simulink model "pv_resource_dynamic_standalone"  (R2024b)
settings: Solver=ode14x  StartTime=0.0  StopTime=1.0  FixedStep=5e-5  RelTol=1e-3
InitFcn:
  | setup_v2_paths; define_resource_buses(true); V2=define_v2_parameters(false); V2.PV.dynamic.enabled=true; V2.PV.filter.topology='LCL';
undefined symbols (not defined in the file): DiscIntNeverNeededParam
libraries: nesl_utility x18, ee_lib x12, fl_lib x11
settings Model: SimulationMode=accelerator  Creator=qyj  LastModifiedBy=qyj

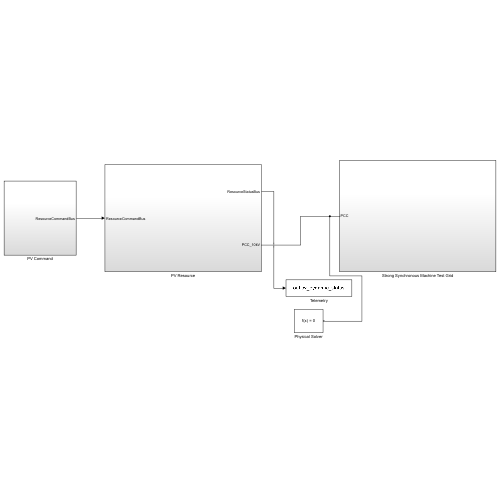
[thumbnail: Simulink's stored preview of the top-level diagram]
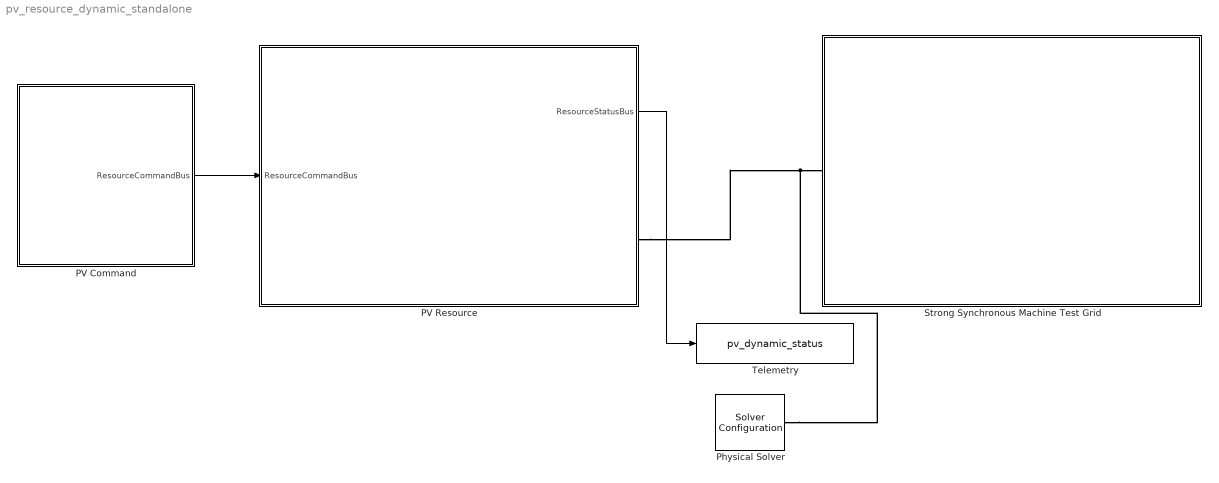
== system pv_resource_dynamic_standalone ==
  PV Command : Subsystem
  PV Resource : Subsystem
  Physical Solver : nesl_utility/Solver Configuration  PhysicalDomain=network_engine_domain  SubClassName=solver  LeftPortType=input  RightPortType=generic  Tones=[]  Harmonics=[]  SimulateNoise=off  Profile=off  UseLocalSampling=off  EnableSwitchedLinearOptims=on  FrequencyDomain=off  UseCCode=off  RelTol=0.001  AbsTol=0.001  MinStep=1e-09  ToWorkspace=off  RevertToSquareIcSolve=off  NumHomotopyIterations=100  PhasorMode=off  PhasorModeNumHarmonics=1  ConsistencySolver=NEWTON_XTOL_AFTER_FTOL  IndexReductionMethod=DerivativeReplacement  DoDC=off  ResidualTolerance=1e-09  ConsistencyTolSource=GLOBAL  ConsistencyAbsTol=0.001  ConsistencyRelTol=0.001  ConsistencyTolFactor=0.001  UseLocalSolver=off  LocalSolverChoice=NE_BACKWARD_EULER_ADVANCER  ResolveIndetEquations=on  FunctionEvalNumThread=1  LocalSolverSampleTime=0.001  DoFixedCost=off  MaxNonlinIter=3  MaxModeIter=2  ComputeImpulses=off  ImpulseIterations=2  LinearAlgebra=auto  LinearAlgebraNumThread=0  EquationFormulation=NE_TIME_EF  DelaysMemoryBudget=1024  AutomaticFiltering=on  FilteringTimeConstant=0.001  PartitionStorageMethod=AS_NEEDED  PartitionMemoryBudget=1024  PartitionMethod=ROBUST  MultibodyUseLocalSolver=off  MultibodyLocalSolverChoice=ODE1  MultibodyLocalSolverSampleTime=0.001
  Strong Synchronous Machine Test Grid : Subsystem
  Telemetry : ToWorkspace  VariableName=pv_dynamic_status  SaveFormat=Timeseries  SampleTime=-1
  wires:
  PV Command/1(ResourceCommandBus) -> PV Resource/1(ResourceCommandBus)
  PV Resource/1(ResourceStatusBus) -> Telemetry/1
  connections:
  PV Resource/RConn1 -- Strong Synchronous Machine Test Grid/LConn1 -- Physical Solver/RConn1

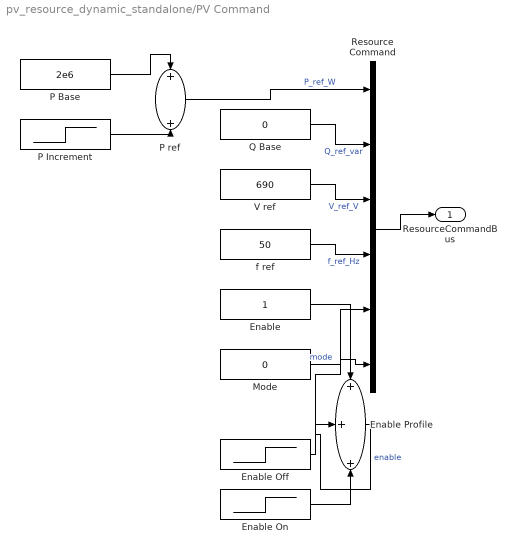
== system pv_resource_dynamic_standalone/PV Command ==
  Enable : Constant
  Enable Off : Step  Time=10  After=-1  SampleTime=0
  Enable On : Step  Time=11  SampleTime=0
  Enable Profile : Sum  Inputs=+++
  Mode : Constant  Value=0
  P Base : Constant  Value=2e6
  P Increment : Step  Time=0.3  After=1e6  SampleTime=0
  P ref : Sum
  Q Base : Constant  Value=0
  Resource Command : BusCreator  Inputs=6  OutDataTypeStr=Bus: ResourceCommandBus
  V ref : Constant  Value=690
  f ref : Constant  Value=50
  ResourceCommandBus : Outport
  wires:
  P Base/1 -> P ref/1
  P Increment/1 -> P ref/2
  Enable/1 -> Enable Profile/1
  Enable Off/1 -> Enable Profile/2
  Enable On/1 -> Enable Profile/3
  P ref/1 -> Resource Command/1  "P_ref_W"
  Q Base/1 -> Resource Command/2  "Q_ref_var"
  V ref/1 -> Resource Command/3  "V_ref_V"
  f ref/1 -> Resource Command/4  "f_ref_Hz"
  Enable Profile/1 -> Resource Command/5  "enable"
  Mode/1 -> Resource Command/6  "mode"
  Resource Command/1 -> ResourceCommandBus/1

== system pv_resource_dynamic_standalone/PV Resource ==
  ResourceCommandBus : Inport
  01 PV Source and DC Side : Subsystem
  02 PCS : Subsystem
  03 AC Interface : Subsystem
      settings: AttributesFormatString=independent filter + 0.69/10 kV transformer + PCC sensing
  Status Interface : Subsystem
  PCC_10kV : PMIOPort  Side=Right  ConnectionType=Connection: foundation.electrical.three_phase
  ResourceStatusBus : Outport  OutDataTypeStr=Bus: ResourceStatusBus
  wires:
  ResourceCommandBus/1 -> 01 PV Source and DC Side/1(Command), 02 PCS/1(Command), Status Interface/4(ResourceCommandBus)
  01 PV Source and DC Side/1(Telemetry) -> 02 PCS/2(DC Telemetry), Status Interface/1(Source)
  03 AC Interface/1(PCCMeasurementBus) -> 02 PCS/3(PCCMeasurementBus), Status Interface/3(PCC)
  02 PCS/1(Telemetry) -> Status Interface/2(PCS)
  Status Interface/1(ResourceStatusBus) -> ResourceStatusBus/1
  connections:
  01 PV Source and DC Side/RConn1 -- 02 PCS/LConn1
  01 PV Source and DC Side/RConn2 -- 02 PCS/LConn2
  02 PCS/RConn1 -- 03 AC Interface/LConn1
  03 AC Interface/RConn1 -- PCC_10kV/RConn1

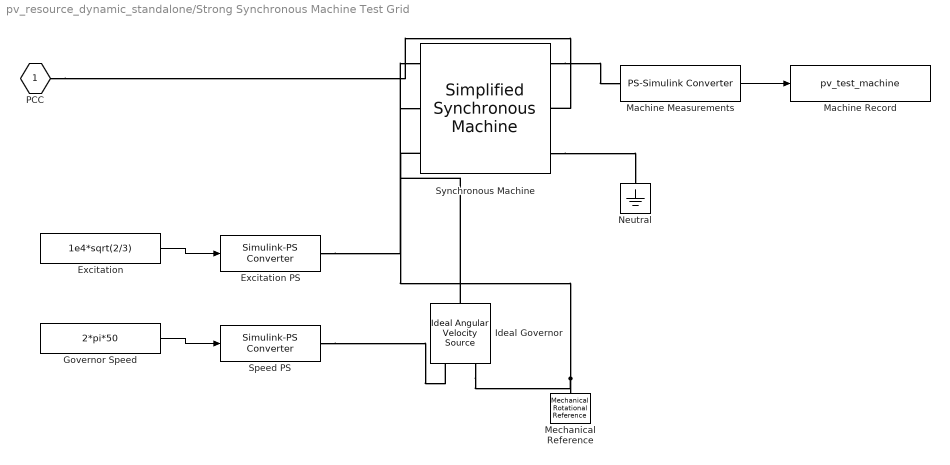
== system pv_resource_dynamic_standalone/Strong Synchronous Machine Test Grid ==
  Excitation : Constant  Value=1e4*sqrt(2/3)
  Excitation PS : nesl_utility/Simulink-PS Converter  PhysicalDomain=network_engine_domain  SubClassName=ps_input  LeftPortType=input  RightPortType=output  PseudoPeriodic=off  Frequencies=[]  NoiseDistribution=none  NoiseParameters=[]  Unit=V  AffineConversion=off  FilteringAndDerivatives=zero  SimscapeFilterOrder=1  InputFilterTimeConstant=0.001  UdotUserProvided=0
  Governor Speed : Constant  Value=2*pi*50
  Ideal Governor : fl_lib/Mechanical/Mechanical Sources/Ideal Angular Velocity Source
  Machine Measurements : nesl_utility/PS-Simulink Converter  PhysicalDomain=network_engine_domain  SubClassName=ps_output  LeftPortType=input  RightPortType=output  PseudoPeriodic=off  Frequencies=[]  VectorFormat=inherit  Unit=1  AffineConversion=off
  Machine Record : ToWorkspace  VariableName=pv_test_machine  SaveFormat=Timeseries  SampleTime=-1
  Mechanical Reference : fl_lib/Mechanical/Rotational Elements/Mechanical Rotational Reference
  Neutral : fl_lib/Electrical/Electrical Elements/Electrical Reference
  Speed PS : nesl_utility/Simulink-PS Converter  PhysicalDomain=network_engine_domain  SubClassName=ps_input  LeftPortType=input  RightPortType=output  PseudoPeriodic=off  Frequencies=[]  NoiseDistribution=none  NoiseParameters=[]  Unit=rad/s  AffineConversion=off  FilteringAndDerivatives=zero  SimscapeFilterOrder=1  InputFilterTimeConstant=0.001  UdotUserProvided=0
  Synchronous Machine : ee_lib/Electromechanical/Synchronous/Simplified Synchronous Machine  port_option=ee.enum.threePhasePort.composite  SRated=100e6 A*V  VRated=10e3 V  FRated=50 Hz  nPolePairs=1  param_unit=ee.enum.unit.si  R_si=0.01 Ohm  L_si=0.001 H  R_pu=0.05  L_pu=0.3  initialization_option=ee.enum.sm.initialization.electrical  source_type=ee.enum.sm.load_flow_source_type.Swing  Vmag0=10e3 V  Vang0=0 deg  Pt0=0 A*V  Qt0=0 A*V  minimum_pu=0.95  phase_search_range=[-inf, inf] deg  gmin=1e-6 S  connection_option=ee.enum.Connection.wye  angular_position_diff_specify=off  angular_position_diff_priority=None  angular_position_diff=0 rad  angular_position_diff_nominal_specify=off  angular_position_diff_nominal_value=1  angular_position_diff_nominal_unit=rad  pu_psid_specify=off  pu_psid_priority=None  pu_psid=0  pu_psid_nominal_specify=off  pu_psid_nominal_value=1  pu_psid_nominal_unit=1  pu_psiq_specify=off  pu_psiq_priority=None  pu_psiq=0  pu_psiq_nominal_specify=off  pu_psiq_nominal_value=1  pu_psiq_nominal_unit=1  pu_psi0_specify=off  pu_psi0_priority=None  pu_psi0=0  pu_psi0_nominal_specify=off  pu_psi0_nominal_value=1  pu_psi0_nominal_unit=1  angular_torque_specify=off  angular_torque_priority=None  angular_torque=0 N*m  angular_torque_nominal_specify=off  angular_torque_nominal_value=1  angular_torque_nominal_unit=N*m  Tmeas=298.15 K  alpha=3.93e-3 1/K  stator_thermal_mass=100 J/K  rotor_thermal_mass=200 J/K  temperatureA_specify=off  temperatureA_priority=High  temperatureA=25 degC  temperatureA_nominal_specify=off  temperatureA_nominal_value=1  temperatureA_nominal_unit=degC  temperatureB_specify=off  temperatureB_priority=High  temperatureB=25 degC  temperatureB_nominal_specify=off  temperatureB_nominal_value=1  temperatureB_nominal_unit=degC  temperatureC_specify=off  temperatureC_priority=High  temperatureC=25 degC  temperatureC_nominal_specify=off  temperatureC_nominal_value=1  temperatureC_nominal_unit=degC  temperatureR_specify=off  temperatureR_priority=High  temperatureR=25 degC  temperatureR_nominal_specify=off  temperatureR_nominal_value=1  temperatureR_nominal_unit=degC
      settings: InternalSimscapePortConfiguration="{\"Bottom\":[],\"Left\":[{\"id\":\"E_si\",\"label\":\"E_si\",\"type\":\"input\"},{\"id\":\"R\",\"label\":\"R\",\"type\":\"foundation.mechanical.rotational.rotational\"},{\"id\":\"C\",\"label\":\"C\",\"type\":\"foundation.mechanical.rotational.rotational\"}],\"Right\":[{\"id\":\"pu_output\",\"label\":\"o\",\"type\":\"output\"},{\"id\":\"N\",\"label\":\"~\",\"type\":\"foundation.electrical.three_phase\"},{\"id\":\"n\",\"label\":\"n\",\"type\":\"foundation.electrical.electrical\"}],\"Top\":[]}"
  PCC : PMIOPort  Side=Left  ConnectionType=Connection: foundation.electrical.three_phase
  wires:
  Excitation/1 -> Excitation PS/1
  Governor Speed/1 -> Speed PS/1
  Machine Measurements/1 -> Machine Record/1
  connections:
  PCC/RConn1 -- Synchronous Machine/RConn2
  Synchronous Machine/RConn3 -- Neutral/LConn1
  Excitation PS/RConn1 -- Synchronous Machine/LConn1
  Speed PS/RConn1 -- Ideal Governor/RConn1
  Ideal Governor/LConn1 -- Synchronous Machine/LConn2
  Mechanical Reference/LConn1 -- Ideal Governor/RConn2 -- Synchronous Machine/LConn3
  Synchronous Machine/RConn1 -- Machine Measurements/LConn1

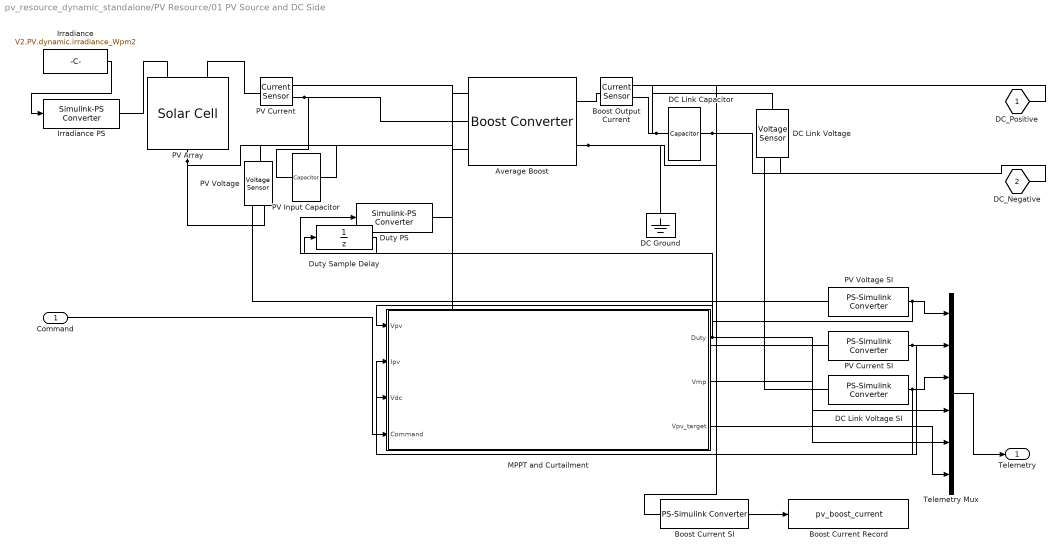
== system pv_resource_dynamic_standalone/PV Resource/01 PV Source and DC Side ==
  Command : Inport
  Average Boost : ee_lib/Semiconductors & Converters/Converters/Boost Converter  port_option=ee.enum.controlport.ps  device_type=ee.enum.converters.switchingdevice.averaged  Vf=0.8 V  Ron=0.001 Ohm  Rds=0.001 Ohm  Goff=1e-5 1/Ohm  Vgt=1 V  Vgt_off=-1 V  Ih=1 A  Vth=6 V  K=0  diode_param=ee.enum.converters.protectiondiode.nodynamics  diode_Vf=0.8 V  diode_Ron=0.001 Ohm  diode_Goff=1e-5 1/Ohm  diode_C=50 nF  diode_iRM=-235 A  diode_iF=300 A  diode_idot=-50 A/us  diode_trr_param=ee.enum.converters.diodetrr.trr_factor  diode_trr_factor=3  diode_trr=15 us  diode_Qrr=1500 s*uA  Lf=V2.PV.dynamic.Lboost_H H  Rl=V2.PV.dynamic.Rboost_ohm Ohm  Cf=1e-6 F  Rf=0.001 Ohm  snubber_type=ee.enum.converters.snubber.exclude  Cs=1e-7 F  Rs=0.1 Ohm  iL_specify=off  iL_priority=High  iL=0 A  iL_nominal_specify=off  iL_nominal_value=1  iL_nominal_unit=A  vc_specify=on  vc_priority=High  vc=V2.PV.dynamic.Vdc_ref_V V  vc_nominal_specify=off  vc_nominal_value=1  vc_nominal_unit=V
      settings: InternalSimscapePortConfiguration="{\"Bottom\":[],\"Left\":[{\"id\":\"G\",\"label\":\"G\",\"type\":\"input\"},{\"id\":\"p1\",\"label\":\"1+\",\"type\":\"foundation.electrical.electrical\"},{\"id\":\"n1\",\"label\":\"1-\",\"type\":\"foundation.electrical.electrical\"}],\"Right\":[{\"id\":\"p2\",\"label\":\"2+\",\"type\":\"foundation.electrical.electrical\"},{\"id\":\"n2\",\"label\":\"2-\",\"type\":\"foundation.electrical.electrical\"}],\"Top\":[]}"
  Boost Current Record : ToWorkspace  VariableName=pv_boost_current  SaveFormat=Timeseries  SampleTime=-1
  Boost Current SI : nesl_utility/PS-Simulink Converter  PhysicalDomain=network_engine_domain  SubClassName=ps_output  LeftPortType=input  RightPortType=output  PseudoPeriodic=off  Frequencies=[]  VectorFormat=inherit  Unit=A  AffineConversion=off
  Boost Output Current : fl_lib/Electrical/Electrical Sensors/Current Sensor
  DC Ground : fl_lib/Electrical/Electrical Elements/Electrical Reference
  DC Link Capacitor : fl_lib/Electrical/Electrical Elements/Capacitor  c=V2.PV.dynamic.Cdc_F F  r=1e-6 Ohm  g=0 1/Ohm  i_specify=off  i_priority=None  i=0 A  i_nominal_specify=off  i_nominal_value=1  i_nominal_unit=A  v_specify=off  v_priority=None  v=0 V  v_nominal_specify=off  v_nominal_value=1  v_nominal_unit=V  vc_specify=on  vc_priority=High  vc=V2.PV.dynamic.Vdc_ref_V V  vc_nominal_specify=off  vc_nominal_value=1  vc_nominal_unit=V
  DC Link Voltage : fl_lib/Electrical/Electrical Sensors/Voltage Sensor
  DC Link Voltage SI : nesl_utility/PS-Simulink Converter  PhysicalDomain=network_engine_domain  SubClassName=ps_output  LeftPortType=input  RightPortType=output  PseudoPeriodic=off  Frequencies=[]  VectorFormat=inherit  Unit=V  AffineConversion=off
  Duty PS : nesl_utility/Simulink-PS Converter  PhysicalDomain=network_engine_domain  SubClassName=ps_input  LeftPortType=input  RightPortType=output  PseudoPeriodic=off  Frequencies=[]  NoiseDistribution=none  NoiseParameters=[]  Unit=1  AffineConversion=off  FilteringAndDerivatives=zero  SimscapeFilterOrder=1  InputFilterTimeConstant=0.001  UdotUserProvided=0
  Duty Sample Delay : UnitDelay  SampleTime=V2.PV.dynamic.sample_s  HasFrameUpgradeWarning=on
  Irradiance : Constant  Value=V2.PV.dynamic.irradiance_Wpm2
  Irradiance PS : nesl_utility/Simulink-PS Converter  PhysicalDomain=network_engine_domain  SubClassName=ps_input  LeftPortType=input  RightPortType=output  PseudoPeriodic=off  Frequencies=[]  NoiseDistribution=none  NoiseParameters=[]  Unit=W/m^2  AffineConversion=off  FilteringAndDerivatives=zero  SimscapeFilterOrder=1  InputFilterTimeConstant=0.001  UdotUserProvided=0
  MPPT and Curtailment : Subsystem
  PV Array : ee_lib/Sources/Solar Cell  prm=ee.enum.sources.solar_cell_prm.datasheet  Isc=V2.PV.dynamic.Isc_cell_A A  Voc=V2.PV.dynamic.Voc_cell_V V  Is=1e-6 A  Is2=0 A  Iph=7.34 A  Ir0=1000 W/m^2  ec=1.5  N2=2  Rs=0 Ohm  Rp=inf Ohm  N_series=V2.PV.dynamic.Nseries  N_parallel=V2.PV.dynamic.Nparallel  TIPH1=0 1/K  EG=1.11 eV  TXIS1=3  TXIS2=3  TRS1=0  TRP1=0  Tmeas=25 degC  TFIXED=V2.PV.dynamic.temperature_degC degC  thermal_mass=100 J/K  initial_temperature=25 degC
  PV Current : fl_lib/Electrical/Electrical Sensors/Current Sensor
  PV Current SI : nesl_utility/PS-Simulink Converter  PhysicalDomain=network_engine_domain  SubClassName=ps_output  LeftPortType=input  RightPortType=output  PseudoPeriodic=off  Frequencies=[]  VectorFormat=inherit  Unit=A  AffineConversion=off
  PV Input Capacitor : fl_lib/Electrical/Electrical Elements/Capacitor  c=V2.PV.dynamic.Cpv_F F  r=1e-6 Ohm  g=0 1/Ohm  i_specify=off  i_priority=None  i=0 A  i_nominal_specify=off  i_nominal_value=1  i_nominal_unit=A  v_specify=off  v_priority=None  v=0 V  v_nominal_specify=off  v_nominal_value=1  v_nominal_unit=V  vc_specify=on  vc_priority=High  vc=V2.PV.dynamic.Vmp_initial_V V  vc_nominal_specify=off  vc_nominal_value=1  vc_nominal_unit=V
  PV Voltage : fl_lib/Electrical/Electrical Sensors/Voltage Sensor
  PV Voltage SI : nesl_utility/PS-Simulink Converter  PhysicalDomain=network_engine_domain  SubClassName=ps_output  LeftPortType=input  RightPortType=output  PseudoPeriodic=off  Frequencies=[]  VectorFormat=inherit  Unit=V  AffineConversion=off
  Telemetry Mux : Mux  Inputs=6
  DC_Positive : PMIOPort  Side=Right  ConnectionType=Connection: foundation.electrical.electrical
  DC_Negative : PMIOPort  Port=2  Side=Right  ConnectionType=Connection: foundation.electrical.electrical
  Telemetry : Outport
  wires:
  Irradiance/1 -> Irradiance PS/1
  PV Voltage SI/1 -> MPPT and Curtailment/1(Vpv), Telemetry Mux/1
  PV Current SI/1 -> MPPT and Curtailment/2(Ipv), Telemetry Mux/2
  DC Link Voltage SI/1 -> MPPT and Curtailment/3(Vdc), Telemetry Mux/3
  Command/1 -> MPPT and Curtailment/4(Command)
  MPPT and Curtailment/1(Duty) -> Duty Sample Delay/1, Telemetry Mux/4
  Duty Sample Delay/1 -> Duty PS/1
  MPPT and Curtailment/2(Vmp) -> Telemetry Mux/5
  MPPT and Curtailment/3(Vpv_target) -> Telemetry Mux/6
  Telemetry Mux/1 -> Telemetry/1
  Boost Current SI/1 -> Boost Current Record/1
  connections:
  Irradiance PS/RConn1 -- PV Array/LConn1
  PV Array/LConn2 -- PV Current/LConn1
  Average Boost/LConn2 -- PV Current/RConn2 -- PV Input Capacitor/LConn1 -- PV Voltage/LConn1
  Average Boost/LConn3 -- PV Array/RConn1 -- PV Voltage/RConn2 -- PV Input Capacitor/RConn1
  Average Boost/RConn1 -- Boost Output Current/LConn1
  Boost Output Current/RConn2 -- DC Link Voltage/LConn1 -- DC Link Capacitor/LConn1 -- DC_Positive/RConn1
  Average Boost/RConn2 -- DC Ground/LConn1 -- DC Link Voltage/RConn2 -- DC Link Capacitor/RConn1 -- DC_Negative/RConn1
  PV Voltage/RConn1 -- PV Voltage SI/LConn1
  PV Current/RConn1 -- PV Current SI/LConn1
  DC Link Voltage/RConn1 -- DC Link Voltage SI/LConn1
  Duty PS/RConn1 -- Average Boost/LConn1
  Boost Output Current/RConn1 -- Boost Current SI/LConn1

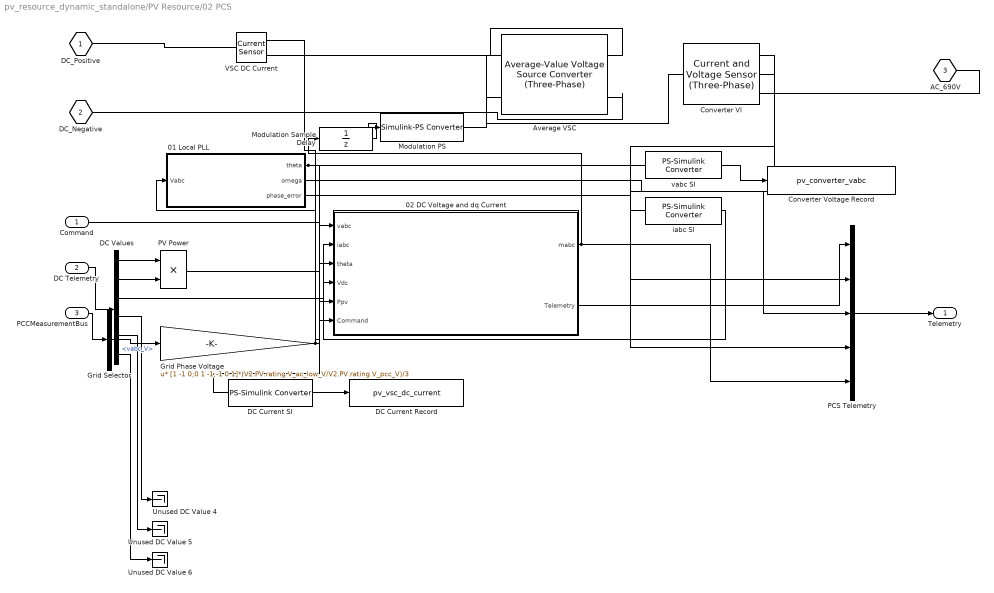
== system pv_resource_dynamic_standalone/PV Resource/02 PCS ==
  Command : Inport
  DC Telemetry : Inport  Port=2
  PCCMeasurementBus : Inport  Port=3
  01 Local PLL : Subsystem
      settings: AttributesFormatString=local PCC voltage only
  02 DC Voltage and dq Current : Subsystem
  Average VSC : ee_lib/Semiconductors & Converters/Converters/Average-Value Voltage Source Converter (Three-Phase)  port_option=ee.enum.threePhasePort.composite  frequency_option=ee.enum.converters.frequency.variable  input_option=ee.enum.converters.inputOption.ModWave  FRated=V2.PV.rating.f_Hz Hz  losses_parameterization=ee.enum.converters.losses.fixed  Pfixed=1 W  ks=0.01  kc1=1.7 V  kc2=0.01 Ohm  Ploss_vect=[100, 800, 1870, 3250, 4900] W  Irms_vect=[10, 100, 200, 300, 400] A  Vdc_nom=V2.PV.dynamic.Vdc_ref_V V  thermal_mass=30000 J/K  temperature_specify=off  temperature_priority=High  temperature=298.15 K  temperature_nominal_specify=off  temperature_nominal_value=1  temperature_nominal_unit=K
      settings: InternalSimscapePortConfiguration="{\"Bottom\":[],\"Left\":[{\"id\":\"ModWave\",\"label\":\"ModWave\",\"type\":\"input\"},{\"id\":\"N\",\"label\":\"~\",\"type\":\"foundation.electrical.three_phase\"}],\"Right\":[{\"id\":\"p\",\"label\":\"+\",\"type\":\"foundation.electrical.electrical\"},{\"id\":\"n\",\"label\":\"-\",\"type\":\"foundation.electrical.electrical\"}],\"Top\":[]}"
  Converter VI : ee_lib/Sensors & Transducers/Current and Voltage Sensor (Three-Phase)  vMeasurementType=ee.enum.vmeasurement.lg  outputUnit=ee.enum.unit.si  SRated=100e6 A*V  VRated=24e3 V  I_specify=off  I_priority=None  I=[0, 0, 0] A  I_nominal_specify=off  I_nominal_value=1  I_nominal_unit=A  V_specify=off  V_priority=None  V=[0, 0, 0] V  V_nominal_specify=off  V_nominal_value=1  V_nominal_unit=V
      settings: InternalSimscapePortConfiguration="{\"Bottom\":[],\"Left\":[{\"id\":\"N1\",\"label\":\"~1\",\"type\":\"foundation.electrical.three_phase\"}],\"Right\":[{\"id\":\"V_output\",\"label\":\"V\",\"type\":\"output\"},{\"id\":\"I_output\",\"label\":\"I\",\"type\":\"output\"},{\"id\":\"N2\",\"label\":\"~2\",\"type\":\"foundation.electrical.three_phase\"}],\"Top\":[]}"
  Converter Voltage Record : ToWorkspace  VariableName=pv_converter_vabc  SaveFormat=Timeseries  SampleTime=-1
  DC Current Record : ToWorkspace  VariableName=pv_vsc_dc_current  SaveFormat=Timeseries  SampleTime=-1
  DC Current SI : nesl_utility/PS-Simulink Converter  PhysicalDomain=network_engine_domain  SubClassName=ps_output  LeftPortType=input  RightPortType=output  PseudoPeriodic=off  Frequencies=[]  VectorFormat=inherit  Unit=A  AffineConversion=off
  DC Values : Demux  Outputs=6
  Grid Phase Voltage : Gain  Gain=[1 -1 0;0 1 -1;-1 0 1]*(V2.PV.rating.V_ac_low_V/V2.PV.rating.V_pcc_V)/3  Multiplication=Matrix(u*K)
  Grid Selector : BusSelector  OutputSignals=vabc_V
  Modulation PS : nesl_utility/Simulink-PS Converter  PhysicalDomain=network_engine_domain  SubClassName=ps_input  LeftPortType=input  RightPortType=output  PseudoPeriodic=off  Frequencies=[]  NoiseDistribution=none  NoiseParameters=[]  Unit=1  AffineConversion=off  FilteringAndDerivatives=zero  SimscapeFilterOrder=1  InputFilterTimeConstant=0.001  UdotUserProvided=0
  Modulation Sample Delay : UnitDelay  InitialCondition=[0;-0.39;0.39]  SampleTime=V2.PV.dynamic.sample_s  HasFrameUpgradeWarning=on
  PCS Telemetry : Mux  Inputs=5
  PV Power : Product
  Unused DC Value 4 : Terminator
  Unused DC Value 5 : Terminator
  Unused DC Value 6 : Terminator
  VSC DC Current : fl_lib/Electrical/Electrical Sensors/Current Sensor
  iabc SI : nesl_utility/PS-Simulink Converter  PhysicalDomain=network_engine_domain  SubClassName=ps_output  LeftPortType=input  RightPortType=output  PseudoPeriodic=off  Frequencies=[]  VectorFormat=inherit  Unit=A  AffineConversion=off
  vabc SI : nesl_utility/PS-Simulink Converter  PhysicalDomain=network_engine_domain  SubClassName=ps_output  LeftPortType=input  RightPortType=output  PseudoPeriodic=off  Frequencies=[]  VectorFormat=inherit  Unit=V  AffineConversion=off
  DC_Positive : PMIOPort  Side=Left  ConnectionType=Connection: foundation.electrical.electrical
  DC_Negative : PMIOPort  Port=2  Side=Left  ConnectionType=Connection: foundation.electrical.electrical
  AC_690V : PMIOPort  Port=3  Side=Right  ConnectionType=Connection: foundation.electrical.three_phase
  Telemetry : Outport
  wires:
  PCCMeasurementBus/1 -> Grid Selector/1
  Grid Selector/1 -> Grid Phase Voltage/1  "<vabc_V>"
  Grid Phase Voltage/1 -> 01 Local PLL/1(Vabc), 02 DC Voltage and dq Current/1(vabc)
  vabc SI/1 -> Converter Voltage Record/1
  DC Telemetry/1 -> DC Values/1
  DC Values/4 -> Unused DC Value 4/1
  DC Values/5 -> Unused DC Value 5/1
  DC Values/6 -> Unused DC Value 6/1
  DC Values/1 -> PV Power/1
  DC Values/2 -> PV Power/2
  iabc SI/1 -> 02 DC Voltage and dq Current/2(iabc)
  01 Local PLL/1(theta) -> 02 DC Voltage and dq Current/3(theta), PCS Telemetry/2
  DC Values/3 -> 02 DC Voltage and dq Current/4(Vdc)
  PV Power/1 -> 02 DC Voltage and dq Current/5(Ppv)
  Command/1 -> 02 DC Voltage and dq Current/6(Command)
  02 DC Voltage and dq Current/1(mabc) -> Modulation Sample Delay/1, PCS Telemetry/5
  Modulation Sample Delay/1 -> Modulation PS/1
  02 DC Voltage and dq Current/2(Telemetry) -> PCS Telemetry/1
  01 Local PLL/2(omega) -> PCS Telemetry/3
  01 Local PLL/3(phase_error) -> PCS Telemetry/4
  PCS Telemetry/1 -> Telemetry/1
  DC Current SI/1 -> DC Current Record/1
  connections:
  DC_Positive/RConn1 -- VSC DC Current/LConn1
  VSC DC Current/RConn2 -- Average VSC/RConn1
  DC_Negative/RConn1 -- Average VSC/RConn2
  Average VSC/LConn2 -- Converter VI/LConn1
  Converter VI/RConn3 -- AC_690V/RConn1
  Converter VI/RConn1 -- vabc SI/LConn1
  Converter VI/RConn2 -- iabc SI/LConn1
  Modulation PS/RConn1 -- Average VSC/LConn1
  VSC DC Current/RConn1 -- DC Current SI/LConn1

== system pv_resource_dynamic_standalone/PV Resource/03 AC Interface ==
  Damped Shunt C : ee_lib/Passive/RLC Assemblies/RLC (Three-Phase)  port_option=ee.enum.threePhasePort.composite  component_structure=ee.enum.rlc.structure.SeriesRC  R=V2.PV.filter.Rd_ohm Ohm  L=1e-3 H  C=V2.PV.filter.C_F F  R_parasitic=0 Ohm  G_parasitic=0 1/Ohm  IL_specify=off  IL_priority=High  IL=[0, 0, 0] A  IL_nominal_specify=off  IL_nominal_value=1  IL_nominal_unit=A  VC_specify=off  VC_priority=High  VC=[0, 0, 0] V  VC_nominal_specify=off  VC_nominal_value=1  VC_nominal_unit=V
      settings: InternalSimscapePortConfiguration="{\"Bottom\":[],\"Left\":[{\"id\":\"N1\",\"label\":\"~1\",\"type\":\"foundation.electrical.three_phase\"}],\"Right\":[{\"id\":\"N2\",\"label\":\"~2\",\"type\":\"foundation.electrical.three_phase\"}],\"Top\":[]}"
  Filter Ground : ee_lib/Connectors & References/Grounded Neutral (Three-Phase)
  Grid-side R2 + L2 : ee_lib/Passive/RLC Assemblies/RLC (Three-Phase)  port_option=ee.enum.threePhasePort.composite  component_structure=ee.enum.rlc.structure.SeriesRL  R=V2.PV.filter.R2_ohm Ohm  L=V2.PV.filter.L2_H H  C=1e-6 F  R_parasitic=0 Ohm  G_parasitic=0 1/Ohm  IL_specify=off  IL_priority=High  IL=[0, 0, 0] A  IL_nominal_specify=off  IL_nominal_value=1  IL_nominal_unit=A  VC_specify=off  VC_priority=High  VC=[0, 0, 0] V  VC_nominal_specify=off  VC_nominal_value=1  VC_nominal_unit=V
      settings: InternalSimscapePortConfiguration="{\"Bottom\":[],\"Left\":[{\"id\":\"N1\",\"label\":\"~1\",\"type\":\"foundation.electrical.three_phase\"}],\"Right\":[{\"id\":\"N2\",\"label\":\"~2\",\"type\":\"foundation.electrical.three_phase\"}],\"Top\":[]}"
  Inverter-side R1 + L1 : ee_lib/Passive/RLC Assemblies/RLC (Three-Phase)  port_option=ee.enum.threePhasePort.composite  component_structure=ee.enum.rlc.structure.SeriesRL  R=V2.PV.filter.R1_ohm Ohm  L=V2.PV.filter.L1_H H  C=1e-6 F  R_parasitic=0 Ohm  G_parasitic=0 1/Ohm  IL_specify=off  IL_priority=High  IL=[0, 0, 0] A  IL_nominal_specify=off  IL_nominal_value=1  IL_nominal_unit=A  VC_specify=off  VC_priority=High  VC=[0, 0, 0] V  VC_nominal_specify=off  VC_nominal_value=1  VC_nominal_unit=V
      settings: InternalSimscapePortConfiguration="{\"Bottom\":[],\"Left\":[{\"id\":\"N1\",\"label\":\"~1\",\"type\":\"foundation.electrical.three_phase\"}],\"Right\":[{\"id\":\"N2\",\"label\":\"~2\",\"type\":\"foundation.electrical.three_phase\"}],\"Top\":[]}"
  PCC Measurement : Subsystem
  Step-up Transformer : ee_lib/Passive/Transformers/Two-Winding Transformer (Three-Phase)  SRated=V2.PV.transformer.S_VA A*V  FRated=V2.PV.rating.f_Hz Hz  Winding1Connection=ee.enum.windingconnection.Yg  VRated1=V2.PV.transformer.V1_V V  Winding2Connection=ee.enum.windingconnection.Yg  VRated2=V2.PV.transformer.V2_V V  CoreType=ee.enum.coretype.threelimb  pu_Rw1=V2.PV.transformer.R_pu/2  pu_Rw2=V2.PV.transformer.R_pu/2  leakage_reactance_option=ee.enum.transformer_leakage.exclude  pu_Xl1=0.05  pu_Xl2=0.05  magnetizing_resistance_option=ee.enum.transformer_magnetizingResistance.exclude  pu_Rm=500  magnetizing_reactance_option=ee.enum.transformer_magnetizingReactance.exclude  saturation_option=ee.enum.transformer_saturation.exclude  pu_Xm=500  current_data=[0, .002, 1, 2]  magnetic_flux_data=[0, 1.2, 1.5, 1.51]  pu_X0=0.5  i1_specify=off  i1_priority=None  i1=[0, 0, 0] A  i1_nominal_specify=off  i1_nominal_value=1  i1_nominal_unit=A  i2_specify=off  i2_priority=None  i2=[0, 0, 0] A  i2_nominal_specify=off  i2_nominal_value=1  i2_nominal_unit=A  phi_specify=off  phi_priority=None  phi=[0, 0, 0]  phi_nominal_specify=off  phi_nominal_value=1  phi_nominal_unit=1  power_dissipated_specify=off  power_dissipated_priority=None  power_dissipated=0 W  power_dissipated_nominal_specify=off  power_dissipated_nominal_value=1  power_dissipated_nominal_unit=W
      settings: InternalSimscapePortConfiguration="{\"Bottom\":[],\"Left\":[{\"id\":\"N1\",\"label\":\"~1\",\"type\":\"foundation.electrical.three_phase\"}],\"Right\":[{\"id\":\"N2\",\"label\":\"~2\",\"type\":\"foundation.electrical.three_phase\"}],\"Top\":[]}"
  PCS AC Terminal : PMIOPort  Side=Left  ConnectionType=Connection: foundation.electrical.three_phase
  PCC_10kV : PMIOPort  Port=2  Side=Right  ConnectionType=Connection: foundation.electrical.three_phase
  PCCMeasurementBus : Outport  OutDataTypeStr=Bus: PCCMeasurementBus
  wires:
  PCC Measurement/1(PCCMeasurementBus) -> PCCMeasurementBus/1
  connections:
  PCS AC Terminal/RConn1 -- Inverter-side R1 + L1/LConn1
  Grid-side R2 + L2/LConn1 -- Inverter-side R1 + L1/RConn1 -- Damped Shunt C/LConn1
  Damped Shunt C/RConn1 -- Filter Ground/LConn1
  Grid-side R2 + L2/RConn1 -- Step-up Transformer/LConn1
  Step-up Transformer/RConn1 -- PCC Measurement/LConn1
  PCC Measurement/RConn1 -- PCC_10kV/RConn1

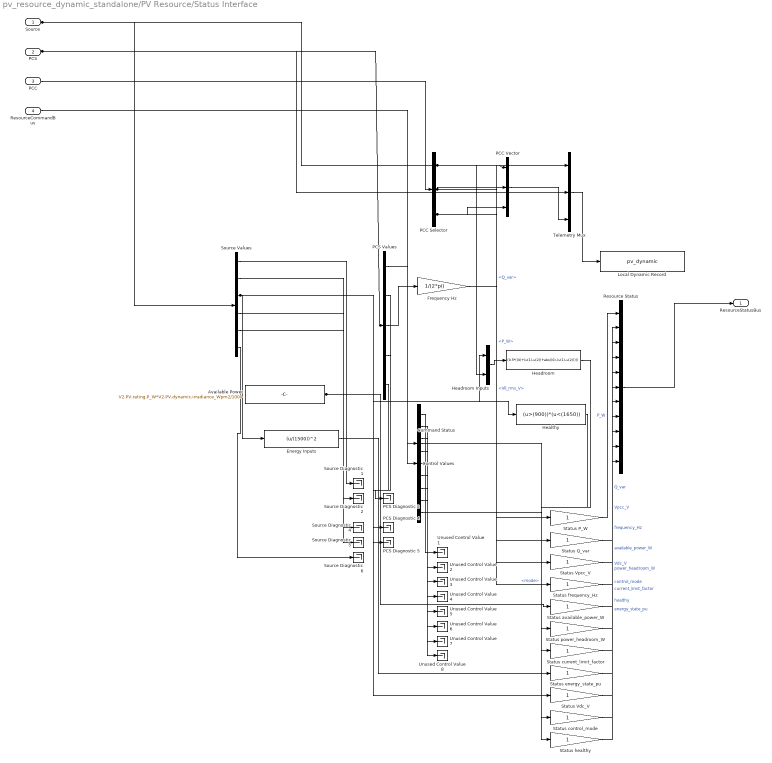
== system pv_resource_dynamic_standalone/PV Resource/Status Interface ==
  Source : Inport
  PCS : Inport  Port=2
  PCC : Inport  Port=3  OutDataTypeStr=Bus: PCCMeasurementBus
  ResourceCommandBus : Inport  Port=4  OutDataTypeStr=Bus: ResourceCommandBus
  Available Power : Constant  Value=V2.PV.rating.P_W*V2.PV.dynamic.irradiance_Wpm2/1000
  Command Status : BusSelector  OutputSignals=mode
  Control Values : Demux  Outputs=9
  Energy Inputs : Fcn  Expr=(u/(1500))^2
  Frequency Hz : Gain  Gain=1/(2*pi)
  Headroom : Fcn  Expr=(0.5*((0)+(u(1)-u(2))+abs((0)-(u(1)-u(2)))))
  Headroom Inputs : Mux  Inputs=2
  Healthy : Fcn  Expr=(u>(900))*(u<(1650))
  Local Dynamic Record : ToWorkspace  VariableName=pv_dynamic  SaveFormat=Timeseries  SampleTime=-1
  PCC Selector : BusSelector  OutputSignals=P_W,Q_var,Vll_rms_V
  PCC Vector : Mux  Inputs=3
  PCS Diagnostic 2 : Terminator
  PCS Diagnostic 4 : Terminator
  PCS Diagnostic 5 : Terminator
  PCS Values : Demux  Outputs=[9 1 1 1 3]
  Resource Status : BusCreator  Inputs=11  OutDataTypeStr=Bus: ResourceStatusBus
  Source Diagnostic {1..2,4..6} (5 alike) : Terminator
  Source Values : Demux  Outputs=6
  Status P_W : Gain
  Status Q_var : Gain
  Status Vdc_V : Gain
  Status Vpcc_V : Gain
  Status available_power_W : Gain
  Status control_mode : Gain
  Status current_limit_factor : Gain
  Status energy_state_pu : Gain
  Status frequency_Hz : Gain
  Status healthy : Gain
  Status power_headroom_W : Gain
  Telemetry Mux : Mux  Inputs=3
  Unused Control Value {1..8} (8 alike) : Terminator
  ResourceStatusBus : Outport  OutDataTypeStr=Bus: ResourceStatusBus
  wires:
  Source/1 -> Telemetry Mux/1, Source Values/1
  PCS/1 -> Telemetry Mux/2, PCS Values/1
  PCC/1 -> PCC Selector/1
  PCC Selector/1 -> PCC Vector/1, Headroom Inputs/2, Status P_W/1  "<P_W>"
  PCC Selector/2 -> PCC Vector/2, Status Q_var/1  "<Q_var>"
  PCC Selector/3 -> PCC Vector/3, Status Vpcc_V/1  "<Vll_rms_V>"
  PCC Vector/1 -> Telemetry Mux/3
  Telemetry Mux/1 -> Local Dynamic Record/1
  PCS Values/3 -> Frequency Hz/1
  Available Power/1 -> Headroom Inputs/1, Status available_power_W/1
  Headroom Inputs/1 -> Headroom/1
  PCS Values/1 -> Control Values/1
  Control Values/1 -> Unused Control Value 1/1
  Control Values/2 -> Unused Control Value 2/1
  Control Values/3 -> Unused Control Value 3/1
  Control Values/4 -> Unused Control Value 4/1
  Control Values/5 -> Unused Control Value 5/1
  Control Values/6 -> Unused Control Value 6/1
  Control Values/7 -> Unused Control Value 7/1
  Control Values/8 -> Unused Control Value 8/1
  Source Values/3 -> Energy Inputs/1, Healthy/1, Status Vdc_V/1
  ResourceCommandBus/1 -> Command Status/1
  Status P_W/1 -> Resource Status/1  "P_W"
  Status Q_var/1 -> Resource Status/2  "Q_var"
  Status Vpcc_V/1 -> Resource Status/3  "Vpcc_V"
  Frequency Hz/1 -> Status frequency_Hz/1
  Status frequency_Hz/1 -> Resource Status/4  "frequency_Hz"
  Status available_power_W/1 -> Resource Status/5  "available_power_W"
  Headroom/1 -> Status power_headroom_W/1
  Status power_headroom_W/1 -> Resource Status/6  "power_headroom_W"
  Control Values/9 -> Status current_limit_factor/1
  Status current_limit_factor/1 -> Resource Status/7  "current_limit_factor"
  Energy Inputs/1 -> Status energy_state_pu/1
  Status energy_state_pu/1 -> Resource Status/8  "energy_state_pu"
  Status Vdc_V/1 -> Resource Status/9  "Vdc_V"
  Command Status/1 -> Status control_mode/1  "<mode>"
  Status control_mode/1 -> Resource Status/10  "control_mode"
  Healthy/1 -> Status healthy/1
  Status healthy/1 -> Resource Status/11  "healthy"
  Resource Status/1 -> ResourceStatusBus/1
  Source Values/1 -> Source Diagnostic 1/1
  Source Values/2 -> Source Diagnostic 2/1
  Source Values/4 -> Source Diagnostic 4/1
  Source Values/5 -> Source Diagnostic 5/1
  Source Values/6 -> Source Diagnostic 6/1
  PCS Values/2 -> PCS Diagnostic 2/1
  PCS Values/4 -> PCS Diagnostic 4/1
  PCS Values/5 -> PCS Diagnostic 5/1

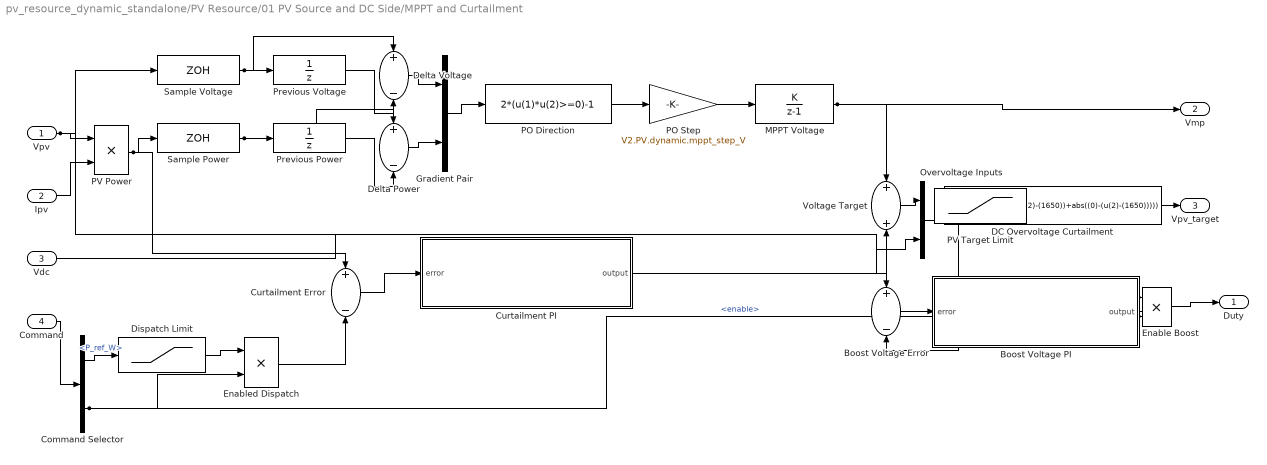
== system pv_resource_dynamic_standalone/PV Resource/01 PV Source and DC Side/MPPT and Curtailment ==
  Vpv : Inport
  Ipv : Inport  Port=2
  Vdc : Inport  Port=3
  Command : Inport  Port=4
  Boost Voltage Error : Sum  Inputs=+-
  Boost Voltage PI : Subsystem
  Command Selector : BusSelector  OutputSignals=P_ref_W,enable
  Curtailment Error : Sum  Inputs=+-
  Curtailment PI : Subsystem
  DC Overvoltage Curtailment : Fcn  Expr=u(1)+2*(0.5*((0)+(u(2)-(1650))+abs((0)-(u(2)-(1650)))))
  Delta Power : Sum  Inputs=+-
  Delta Voltage : Sum  Inputs=+-
  Dispatch Limit : Saturate  UpperLimit=V2.PV.rating.P_W  LowerLimit=0
  Enable Boost : Product
  Enabled Dispatch : Product
  Gradient Pair : Mux  Inputs=2
  MPPT Voltage : DiscreteIntegrator  IntegratorMethod=Accumulation: Forward Euler  gainval=1  InitialCondition=V2.PV.dynamic.Vmp_initial_V  SampleTime=V2.PV.dynamic.mppt_period_s  LimitOutput=on  UpperSaturationLimit=970  LowerSaturationLimit=V2.PV.dynamic.Vpv_min_V  ICPrevOutput=DiscIntNeverNeededParam  ICPrevScaledInput=DiscIntNeverNeededParam
  Overvoltage Inputs : Mux  Inputs=2
  PO Direction : Fcn  Expr=2*(u(1)*u(2)>=0)-1
  PO Step : Gain  Gain=V2.PV.dynamic.mppt_step_V
  PV Power : Product
  PV Target Limit : Saturate  UpperLimit=V2.PV.dynamic.Vpv_max_V  LowerLimit=V2.PV.dynamic.Vpv_min_V
  Previous Power : UnitDelay  SampleTime=V2.PV.dynamic.mppt_period_s  HasFrameUpgradeWarning=on
  Previous Voltage : UnitDelay  InitialCondition=V2.PV.dynamic.Vmp_initial_V  SampleTime=V2.PV.dynamic.mppt_period_s  HasFrameUpgradeWarning=on
  Sample Power : ZeroOrderHold  SampleTime=V2.PV.dynamic.mppt_period_s
  Sample Voltage : ZeroOrderHold  SampleTime=V2.PV.dynamic.mppt_period_s
  Voltage Target : Sum
  Duty : Outport
  Vmp : Outport  Port=2
  Vpv_target : Outport  Port=3
  wires:
  Command/1 -> Command Selector/1
  Command Selector/1 -> Dispatch Limit/1  "<P_ref_W>"
  Dispatch Limit/1 -> Enabled Dispatch/1
  Command Selector/2 -> Enabled Dispatch/2, Enable Boost/2  "<enable>"
  Vpv/1 -> PV Power/1, Sample Voltage/1, Boost Voltage Error/1
  Ipv/1 -> PV Power/2
  PV Power/1 -> Sample Power/1, Curtailment Error/1
  Sample Voltage/1 -> Previous Voltage/1, Delta Voltage/1
  Sample Power/1 -> Previous Power/1, Delta Power/1
  Previous Voltage/1 -> Delta Voltage/2
  Previous Power/1 -> Delta Power/2
  Delta Voltage/1 -> Gradient Pair/1
  Delta Power/1 -> Gradient Pair/2
  Gradient Pair/1 -> PO Direction/1
  PO Direction/1 -> PO Step/1
  PO Step/1 -> MPPT Voltage/1
  Enabled Dispatch/1 -> Curtailment Error/2
  Curtailment Error/1 -> Curtailment PI/1(error)
  MPPT Voltage/1 -> Voltage Target/1, Vmp/1
  Curtailment PI/1(output) -> Voltage Target/2
  Voltage Target/1 -> Overvoltage Inputs/1
  Vdc/1 -> Overvoltage Inputs/2
  Overvoltage Inputs/1 -> DC Overvoltage Curtailment/1
  DC Overvoltage Curtailment/1 -> PV Target Limit/1
  PV Target Limit/1 -> Boost Voltage Error/2, Vpv_target/1
  Boost Voltage Error/1 -> Boost Voltage PI/1(error)
  Boost Voltage PI/1(output) -> Enable Boost/1
  Enable Boost/1 -> Duty/1

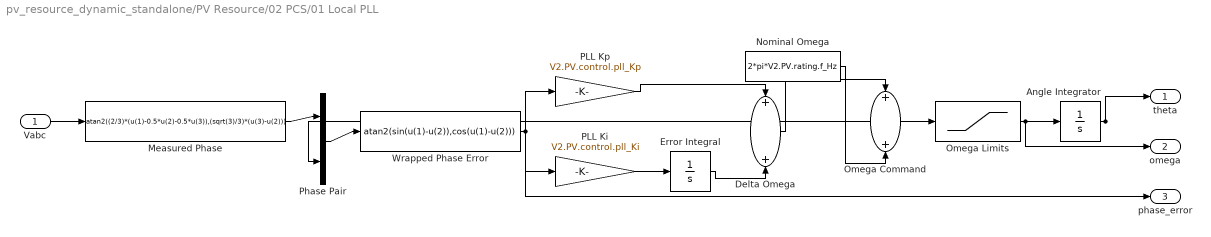
== system pv_resource_dynamic_standalone/PV Resource/02 PCS/01 Local PLL ==
  Vabc : Inport
  Angle Integrator : Integrator  InitialCondition=V2.PV.control.pll_theta0_rad
  Delta Omega : Sum
  Error Integral : Integrator
  Measured Phase : Fcn  Expr=atan2((2/3)*(u(1)-0.5*u(2)-0.5*u(3)),(sqrt(3)/3)*(u(3)-u(2)))
  Nominal Omega : Constant  Value=2*pi*V2.PV.rating.f_Hz
  Omega Command : Sum
  Omega Limits : Saturate  UpperLimit=2*pi*V2.PV.control.pll_max_Hz  LowerLimit=2*pi*V2.PV.control.pll_min_Hz
  PLL Ki : Gain  Gain=V2.PV.control.pll_Ki
  PLL Kp : Gain  Gain=V2.PV.control.pll_Kp
  Phase Pair : Mux  Inputs=2
  Wrapped Phase Error : Fcn  Expr=atan2(sin(u(1)-u(2)),cos(u(1)-u(2)))
  theta : Outport
  omega : Outport  Port=2
  phase_error : Outport  Port=3
  wires:
  Vabc/1 -> Measured Phase/1
  Measured Phase/1 -> Phase Pair/1
  Angle Integrator/1 -> Phase Pair/2, theta/1
  Phase Pair/1 -> Wrapped Phase Error/1
  Wrapped Phase Error/1 -> PLL Kp/1, PLL Ki/1, phase_error/1
  PLL Ki/1 -> Error Integral/1
  PLL Kp/1 -> Delta Omega/1
  Error Integral/1 -> Delta Omega/2
  Delta Omega/1 -> Omega Command/1
  Nominal Omega/1 -> Omega Command/2
  Omega Command/1 -> Omega Limits/1
  Omega Limits/1 -> Angle Integrator/1, omega/1

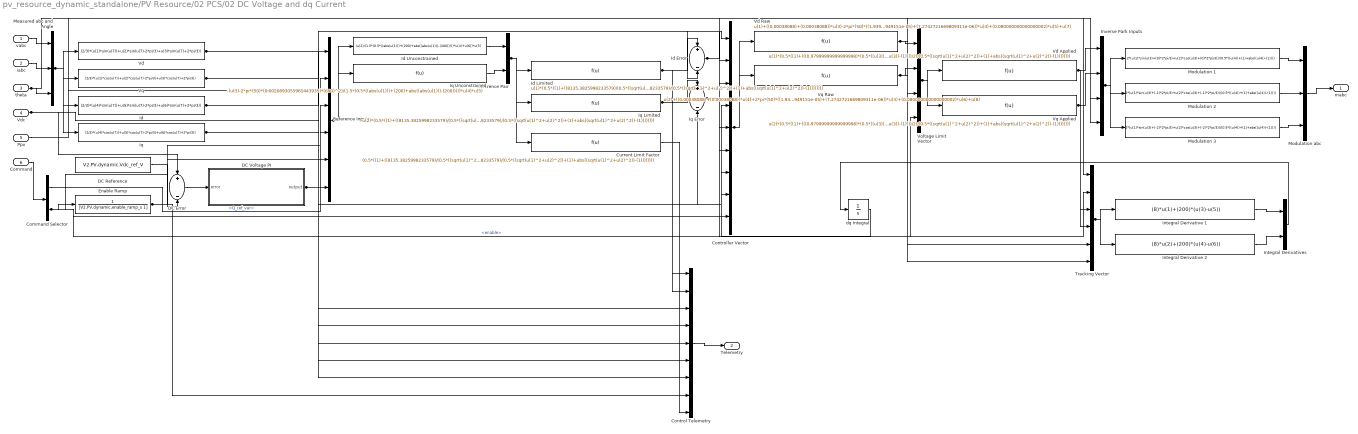
== system pv_resource_dynamic_standalone/PV Resource/02 PCS/02 DC Voltage and dq Current ==
  vabc : Inport
  iabc : Inport  Port=2
  theta : Inport  Port=3
  Vdc : Inport  Port=4
  Ppv : Inport  Port=5
  Command : Inport  Port=6
  Command Selector : BusSelector  OutputSignals=Q_ref_var,enable
  Control Telemetry : Mux  Inputs=9
  Controller Vector : Mux  Inputs=9
  Current Limit Factor : Fcn  Expr=(0.5*((1)+((8135.3825998233579)/(0.5*((sqrt(u(1)^2+u(2)^2))+(1)+abs((sqrt(u(1)^2+u(2)^2))-(1)))))-abs((1)-((8135.3825998233579)/(0.5*((sqrt(u(1)^2+u(2)^2))+(1)+abs((sqrt(u(1)^2+u(2)^2))-(1))))))))
  DC Error : Sum  Inputs=+-
  DC Reference : Constant  Value=V2.PV.dynamic.Vdc_ref_V
  DC Voltage PI : Subsystem
  Enable Ramp : TransferFcn  Numerator=1  Denominator=[V2.PV.dynamic.enable_ramp_s 1]
  Id : Fcn  Expr=(2/3)*(u(4)*sin(u(7))+u(5)*sin(u(7)-2*pi/3)+u(6)*sin(u(7)+2*pi/3))
  Id Error : Sum  Inputs=+-
  Id Limited : Fcn  Expr=u(1)*(0.5*((1)+((8135.3825998233579)/(0.5*((sqrt(u(1)^2+u(2)^2))+(1)+abs((sqrt(u(1)^2+u(2)^2))-(1)))))-abs((1)-((8135.3825998233579)/(0.5*((sqrt(u(1)^2+u(2)^2))+(1)+abs((sqrt(u(1)^2+u(2)^2))-(1))))))))
  Id Unconstrained : Fcn  Expr=(u(2)/(1.5*(0.5*((abs(u(1)))+(200)+abs((abs(u(1)))-(200)))))*u(4)+u(6))*u(5)
  Integral Derivative 1 : Fcn  Expr=(8)*u(1)+(200)*(u(3)-u(5))
  Integral Derivative 2 : Fcn  Expr=(8)*u(2)+(200)*(u(4)-u(6))
  Integral Derivatives : Mux  Inputs=2
  Inverse Park Inputs : Mux
  Iq : Fcn  Expr=(2/3)*(u(4)*cos(u(7))+u(5)*cos(u(7)-2*pi/3)+u(6)*cos(u(7)+2*pi/3))
  Iq Error : Sum  Inputs=+-
  Iq Limited : Fcn  Expr=u(2)*(0.5*((1)+((8135.3825998233579)/(0.5*((sqrt(u(1)^2+u(2)^2))+(1)+abs((sqrt(u(1)^2+u(2)^2))-(1)))))-abs((1)-((8135.3825998233579)/(0.5*((sqrt(u(1)^2+u(2)^2))+(1)+abs((sqrt(u(1)^2+u(2)^2))-(1))))))))
  Iq Unconstrained : Fcn  Expr=-(u(3)-2*pi*(50)*(0.0020893055961443935)*(690)^2)/(1.5*(0.5*((abs(u(1)))+(200)+abs((abs(u(1)))-(200)))))*u(4)*u(5)
  Measured abc and Angle : Mux  Inputs=3
  Modulation 1 : Fcn  Expr=2*(u(1)*sin(u(3)+(0)*2*pi/3)+u(2)*cos(u(3)+(0)*2*pi/3))/(0.5*((u(4))+(1)+abs((u(4))-(1))))
  Modulation 2 : Fcn  Expr=2*(u(1)*sin(u(3)+(-1)*2*pi/3)+u(2)*cos(u(3)+(-1)*2*pi/3))/(0.5*((u(4))+(1)+abs((u(4))-(1))))
  Modulation 3 : Fcn  Expr=2*(u(1)*sin(u(3)+(-2)*2*pi/3)+u(2)*cos(u(3)+(-2)*2*pi/3))/(0.5*((u(4))+(1)+abs((u(4))-(1))))
  Modulation abc : Mux  Inputs=3
  Reference Inputs : Mux  Inputs=6
  Reference Pair : Mux  Inputs=2
  Tracking Vector : Mux  Inputs=6
  Vd : Fcn  Expr=(2/3)*(u(1)*sin(u(7))+u(2)*sin(u(7)-2*pi/3)+u(3)*sin(u(7)+2*pi/3))
  Vd Applied : Fcn  Expr=u(1)*(0.5*((1)+(((0.97999999999999998)*(0.5*((u(3))+(1)+abs((u(3))-(1))))/2)/(0.5*((sqrt(u(1)^2+u(2)^2))+(1)+abs((sqrt(u(1)^2+u(2)^2))-(1)))))-abs((1)-(((0.97999999999999998)*(0.5*((u(3))+(1)+abs((u(3))-(1))))/2)/(0.5*((sqrt(u(1)^2+u(2)^2))+(1)+abs((sqrt(u(1)^2+u(2)^2))-(1))))))))
  Vd Raw : Fcn  Expr=u(1)+((0.00038088)+(0.00038088))*u(3)-2*pi*(50)*((1.9398059111949151e-05)+(7.2742721669809311e-06))*u(4)+(0.080000000000000002)*u(5)+u(7)
  Voltage Limit Vector : Mux
  Vq : Fcn  Expr=(2/3)*(u(1)*cos(u(7))+u(2)*cos(u(7)-2*pi/3)+u(3)*cos(u(7)+2*pi/3))
  Vq Applied : Fcn  Expr=u(2)*(0.5*((1)+(((0.97999999999999998)*(0.5*((u(3))+(1)+abs((u(3))-(1))))/2)/(0.5*((sqrt(u(1)^2+u(2)^2))+(1)+abs((sqrt(u(1)^2+u(2)^2))-(1)))))-abs((1)-(((0.97999999999999998)*(0.5*((u(3))+(1)+abs((u(3))-(1))))/2)/(0.5*((sqrt(u(1)^2+u(2)^2))+(1)+abs((sqrt(u(1)^2+u(2)^2))-(1))))))))
  Vq Raw : Fcn  Expr=u(2)+((0.00038088)+(0.00038088))*u(4)+2*pi*(50)*((1.9398059111949151e-05)+(7.2742721669809311e-06))*u(3)+(0.080000000000000002)*u(6)+u(8)
  dq Integral : Integrator  InitialCondition=[0;0]
  mabc : Outport
  Telemetry : Outport  Port=2
  wires:
  vabc/1 -> Measured abc and Angle/1
  iabc/1 -> Measured abc and Angle/2
  theta/1 -> Measured abc and Angle/3, Inverse Park Inputs/3
  Measured abc and Angle/1 -> Vd/1, Vq/1, Id/1, Iq/1
  Command/1 -> Command Selector/1
  Command Selector/2 -> Enable Ramp/1, Reference Inputs/5, Controller Vector/9, Voltage Limit Vector/4  "<enable>"
  Vdc/1 -> DC Error/1, Controller Vector/8, Voltage Limit Vector/3, Inverse Park Inputs/4
  DC Reference/1 -> DC Error/2
  DC Error/1 -> DC Voltage PI/1(error)
  Vd/1 -> Reference Inputs/1, Controller Vector/1, Control Telemetry/5
  Ppv/1 -> Reference Inputs/2
  Command Selector/1 -> Reference Inputs/3  "<Q_ref_var>"
  Enable Ramp/1 -> Reference Inputs/4, Control Telemetry/8
  DC Voltage PI/1(output) -> Reference Inputs/6, Control Telemetry/7
  Reference Inputs/1 -> Id Unconstrained/1, Iq Unconstrained/1
  Id Unconstrained/1 -> Reference Pair/1
  Iq Unconstrained/1 -> Reference Pair/2
  Reference Pair/1 -> Current Limit Factor/1, Id Limited/1, Iq Limited/1
  Id Limited/1 -> Id Error/1, Control Telemetry/1
  Id/1 -> Id Error/2, Controller Vector/3, Control Telemetry/3
  Iq Limited/1 -> Iq Error/1, Control Telemetry/2
  Iq/1 -> Iq Error/2, Controller Vector/4, Control Telemetry/4
  Vq/1 -> Controller Vector/2, Control Telemetry/6
  Id Error/1 -> Controller Vector/5, Tracking Vector/1
  Iq Error/1 -> Controller Vector/6, Tracking Vector/2
  dq Integral/1 -> Controller Vector/7
  Controller Vector/1 -> Vd Raw/1, Vq Raw/1
  Vd Raw/1 -> Voltage Limit Vector/1, Tracking Vector/5
  Vq Raw/1 -> Voltage Limit Vector/2, Tracking Vector/6
  Voltage Limit Vector/1 -> Vd Applied/1, Vq Applied/1
  Vd Applied/1 -> Tracking Vector/3, Inverse Park Inputs/1
  Vq Applied/1 -> Tracking Vector/4, Inverse Park Inputs/2
  Tracking Vector/1 -> Integral Derivative 1/1, Integral Derivative 2/1
  Integral Derivative 1/1 -> Integral Derivatives/1
  Integral Derivative 2/1 -> Integral Derivatives/2
  Integral Derivatives/1 -> dq Integral/1
  Inverse Park Inputs/1 -> Modulation 1/1, Modulation 2/1, Modulation 3/1
  Modulation 1/1 -> Modulation abc/1
  Modulation 2/1 -> Modulation abc/2
  Modulation 3/1 -> Modulation abc/3
  Modulation abc/1 -> mabc/1
  Current Limit Factor/1 -> Control Telemetry/9
  Control Telemetry/1 -> Telemetry/1

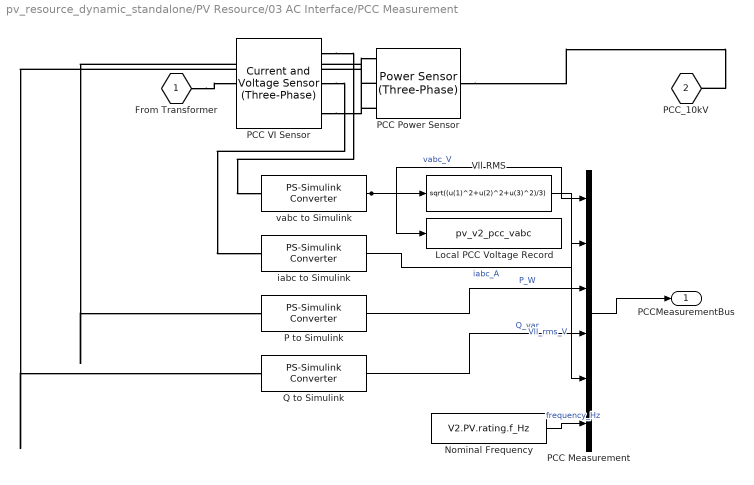
== system pv_resource_dynamic_standalone/PV Resource/03 AC Interface/PCC Measurement ==
  Local PCC Voltage Record : ToWorkspace  VariableName=pv_v2_pcc_vabc  SampleTime=-1
  Nominal Frequency : Constant  Value=V2.PV.rating.f_Hz
  P to Simulink : nesl_utility/PS-Simulink Converter  PhysicalDomain=network_engine_domain  SubClassName=ps_output  LeftPortType=input  RightPortType=output  PseudoPeriodic=off  Frequencies=[]  VectorFormat=inherit  Unit=W  AffineConversion=off
  PCC Measurement : BusCreator  Inputs=6  OutDataTypeStr=Bus: PCCMeasurementBus
  PCC Power Sensor : ee_lib/Sensors & Transducers/Power Sensor (Three-Phase)  load_type=ee.enum.passive.type_balanced.balanced  f0=60 Hz
      settings: InternalSimscapePortConfiguration="{\"Bottom\":[],\"Left\":[{\"id\":\"N1\",\"label\":\"~1\",\"type\":\"foundation.electrical.three_phase\"}],\"Right\":[{\"id\":\"N2\",\"label\":\"~2\",\"type\":\"foundation.electrical.three_phase\"}],\"Top\":[{\"id\":\"Pm\",\"label\":\"P\",\"type\":\"output\"},{\"id\":\"Qm\",\"label\":\"Q\",\"type\":\"output\"}]}"
  PCC VI Sensor : ee_lib/Sensors & Transducers/Current and Voltage Sensor (Three-Phase)  vMeasurementType=ee.enum.vmeasurement.ll  outputUnit=ee.enum.unit.si  SRated=100e6 A*V  VRated=24e3 V  I_specify=off  I_priority=None  I=[0, 0, 0] A  I_nominal_specify=off  I_nominal_value=1  I_nominal_unit=A  V_specify=off  V_priority=None  V=[0, 0, 0] V  V_nominal_specify=off  V_nominal_value=1  V_nominal_unit=V
      settings: InternalSimscapePortConfiguration="{\"Bottom\":[],\"Left\":[{\"id\":\"N1\",\"label\":\"~1\",\"type\":\"foundation.electrical.three_phase\"}],\"Right\":[{\"id\":\"V_output\",\"label\":\"V\",\"type\":\"output\"},{\"id\":\"I_output\",\"label\":\"I\",\"type\":\"output\"},{\"id\":\"N2\",\"label\":\"~2\",\"type\":\"foundation.electrical.three_phase\"}],\"Top\":[]}"
  Q to Simulink : nesl_utility/PS-Simulink Converter  PhysicalDomain=network_engine_domain  SubClassName=ps_output  LeftPortType=input  RightPortType=output  PseudoPeriodic=off  Frequencies=[]  VectorFormat=inherit  Unit=W  AffineConversion=off
  Vll RMS : Fcn  Expr=sqrt((u(1)^2+u(2)^2+u(3)^2)/3)
  iabc to Simulink : nesl_utility/PS-Simulink Converter  PhysicalDomain=network_engine_domain  SubClassName=ps_output  LeftPortType=input  RightPortType=output  PseudoPeriodic=off  Frequencies=[]  VectorFormat=inherit  Unit=A  AffineConversion=off
  vabc to Simulink : nesl_utility/PS-Simulink Converter  PhysicalDomain=network_engine_domain  SubClassName=ps_output  LeftPortType=input  RightPortType=output  PseudoPeriodic=off  Frequencies=[]  VectorFormat=inherit  Unit=V  AffineConversion=off
  From Transformer : PMIOPort  Side=Left  ConnectionType=Connection: foundation.electrical.three_phase
  PCC_10kV : PMIOPort  Port=2  Side=Right  ConnectionType=Connection: foundation.electrical.three_phase
  PCCMeasurementBus : Outport  OutDataTypeStr=Bus: PCCMeasurementBus
  wires:
  vabc to Simulink/1 -> Vll RMS/1, Local PCC Voltage Record/1, PCC Measurement/1  "vabc_V"
  iabc to Simulink/1 -> PCC Measurement/2  "iabc_A"
  P to Simulink/1 -> PCC Measurement/3  "P_W"
  Q to Simulink/1 -> PCC Measurement/4  "Q_var"
  Vll RMS/1 -> PCC Measurement/5  "Vll_rms_V"
  Nominal Frequency/1 -> PCC Measurement/6  "frequency_Hz"
  PCC Measurement/1 -> PCCMeasurementBus/1
  connections:
  From Transformer/RConn1 -- PCC VI Sensor/LConn1
  PCC VI Sensor/RConn3 -- PCC Power Sensor/LConn1
  PCC Power Sensor/RConn1 -- PCC_10kV/RConn1
  PCC VI Sensor/RConn1 -- vabc to Simulink/LConn1
  PCC VI Sensor/RConn2 -- iabc to Simulink/LConn1
  PCC Power Sensor/LConn2 -- P to Simulink/LConn1
  PCC Power Sensor/LConn3 -- Q to Simulink/LConn1

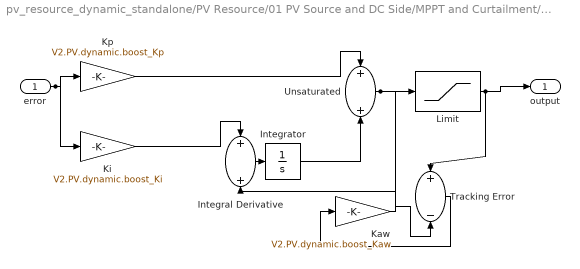
== system pv_resource_dynamic_standalone/PV Resource/01 PV Source and DC Side/MPPT and Curtailment/Boost Voltage PI ==
  error : Inport
  Integral Derivative : Sum
  Integrator : Integrator  InitialCondition=0.4
  Kaw : Gain  Gain=V2.PV.dynamic.boost_Kaw
  Ki : Gain  Gain=V2.PV.dynamic.boost_Ki
  Kp : Gain  Gain=V2.PV.dynamic.boost_Kp
  Limit : Saturate  UpperLimit=V2.PV.dynamic.duty_max  LowerLimit=V2.PV.dynamic.duty_min
  Tracking Error : Sum  Inputs=+-
  Unsaturated : Sum
  output : Outport
  wires:
  error/1 -> Kp/1, Ki/1
  Ki/1 -> Integral Derivative/1
  Kaw/1 -> Integral Derivative/2
  Integral Derivative/1 -> Integrator/1
  Integrator/1 -> Unsaturated/2
  Kp/1 -> Unsaturated/1
  Unsaturated/1 -> Limit/1, Tracking Error/2
  Limit/1 -> output/1, Tracking Error/1
  Tracking Error/1 -> Kaw/1

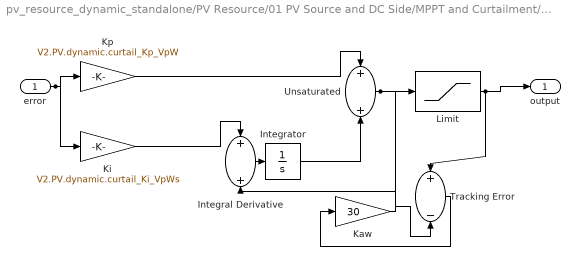
== system pv_resource_dynamic_standalone/PV Resource/01 PV Source and DC Side/MPPT and Curtailment/Curtailment PI ==
  error : Inport
  Integral Derivative : Sum
  Integrator : Integrator  InitialCondition=min(180,V2.PV.dynamic.Vpv_max_V-V2.PV.dynamic.Vmp_initial_V)
  Kaw : Gain  Gain=30
  Ki : Gain  Gain=V2.PV.dynamic.curtail_Ki_VpWs
  Kp : Gain  Gain=V2.PV.dynamic.curtail_Kp_VpW
  Limit : Saturate  UpperLimit=400  LowerLimit=0
  Tracking Error : Sum  Inputs=+-
  Unsaturated : Sum
  output : Outport
  wires:
  error/1 -> Kp/1, Ki/1
  Ki/1 -> Integral Derivative/1
  Kaw/1 -> Integral Derivative/2
  Integral Derivative/1 -> Integrator/1
  Integrator/1 -> Unsaturated/2
  Kp/1 -> Unsaturated/1
  Unsaturated/1 -> Limit/1, Tracking Error/2
  Limit/1 -> output/1, Tracking Error/1
  Tracking Error/1 -> Kaw/1

== system pv_resource_dynamic_standalone/PV Resource/02 PCS/02 DC Voltage and dq Current/DC Voltage PI ==
  error : Inport
  Integral Derivative : Sum
  Integrator : Integrator
  Kaw : Gain  Gain=V2.PV.dynamic.dc_Kaw
  Ki : Gain  Gain=V2.PV.dynamic.dc_Ki_ApVs
  Kp : Gain  Gain=V2.PV.dynamic.dc_Kp_ApV
  Limit : Saturate  UpperLimit=V2.PV.control.Ilimit_peak_A  LowerLimit=-V2.PV.control.Ilimit_peak_A
  Tracking Error : Sum  Inputs=+-
  Unsaturated : Sum
  output : Outport
  wires:
  error/1 -> Kp/1, Ki/1
  Ki/1 -> Integral Derivative/1
  Kaw/1 -> Integral Derivative/2
  Integral Derivative/1 -> Integrator/1
  Integrator/1 -> Unsaturated/2
  Kp/1 -> Unsaturated/1
  Unsaturated/1 -> Limit/1, Tracking Error/2
  Limit/1 -> output/1, Tracking Error/1
  Tracking Error/1 -> Kaw/1
